simulink model "tip_assist_lib_support_pfw_latch_concepting"  (Simulink 9.0)
settings: Solver=VariableStepAuto  StartTime=0.0  StopTime=10.0  RelTol=1e-3
settings Model: Creator=CurriSD  LastModifiedBy=CurriSD
settings DataIOCC: SaveFormat=Dataset
settings OptimizationCC: LifeSpan=auto
settings DebuggingCC: UnderspecifiedInitializationDetection=Simplified  MergeDetectMultiDrivingBlocksExec=error  SFUnexpectedBacktrackingDiag=error  SFNoUnconditionalDefaultTransitionDiag=error  SFExecutionAtInitializationDiag=warning
settings HardwareCC: ProdBitPerPointer=64  ProdBitPerSizeT=64  ProdBitPerPtrDiffT=64  ProdLargestAtomicFloat=Float  ProdIntDivRoundTo=Zero  ProdEndianess=LittleEndian  ProdWordSize=64  ProdHWDeviceType=Intel->x86-64 (Windows64)
settings ModelReferenceCC: PropagateSignalLabelsOutOfModel=on
settings CodeAppCC: StateflowObjectComments=off
settings GRTTargetCC: TargetLangStandard=C99 (ISO)
settings ConfigComp: CovMetricSettings=dwe  CovHtmlReporting=off  CovSaveCumulativeToWorkspaceVar=off  CovSaveSingleToWorkspaceVar=off  CovExternalEMLEnable=on

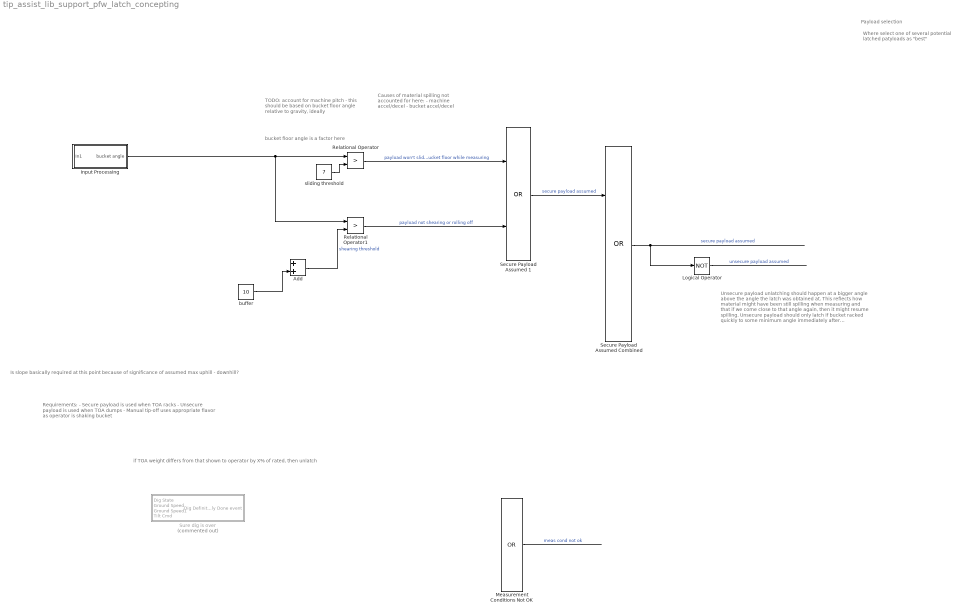
== system tip_assist_lib_support_pfw_latch_concepting ==
  note: if TOA weight differs from that shown to operator by X% of rated, then unlatch
  note: Is slope basically required at this point because of significance of assumed max uphill - downhill?
  note: Unsecure payload unlatching should happen at a bigger angle above the angle the latch was obtained at.  This reflects how material might have been still spilling when measuring and that if we come close to that angle again, then it might resume spilling.
      |
      | Unsecure payload should only latch if bucket racked quickly to some minimum angle immediately after measurement.  Otherwise, payload could still be falling out.
  note: Where select one of several potential latched patyloads as "best"
  note: Payload selection
  note: Requirements:
      | - Secure payload is used when TOA racks
      | - Unsecure payload is used when TOA dumps
      | - Manual tip-off uses appropriate flavor as operator is shaking bucket
  note: bucket floor angle is a factor here
  note: Causes of material spilling not accounted for here:
      | - machine accel/decel
      | - bucket accel/decel
  note: TODO: account for machine pitch - this should be based on bucket floor angle relative to gravity, ideally
  Add : Sum
  Input Processing : Subsystem
  Logical Operator : Logic  Operator=NOT  AllPortsSameDT=off  OutDataTypeStr=boolean
  Measurement Conditions Not OK : Logic  Operator=OR  Inputs=5  AllPortsSameDT=off  OutDataTypeStr=boolean
  Relational Operator : RelationalOperator  Operator=>  OutDataTypeStr=boolean  RndMeth=Simplest
  Relational Operator1 : RelationalOperator  Operator=>  OutDataTypeStr=boolean  RndMeth=Simplest
  Secure Payload Assumed 1 : Logic  Operator=OR  AllPortsSameDT=off  OutDataTypeStr=boolean
  Secure Payload Assumed Combined : Logic  Operator=OR  AllPortsSameDT=off  OutDataTypeStr=boolean
  Sure dig is over : Subsystem  Commented=on
  buffer : Constant  Value=10
  sliding threshold : Constant  Value=7
  wires:
  Measurement Conditions Not OK/1 -> ?  "meas cond not ok"
  Secure Payload Assumed Combined/1 -> Logical Operator/1  "secure payload assumed"
  Logical Operator/1 -> ?  "unsecure payload assumed"
  Relational Operator/1 -> Secure Payload Assumed 1/1  "payload won't slide out against bucket floor while measuring"
  Input Processing/1(bucket angle) -> Relational Operator1/1, Relational Operator/1
  sliding threshold/1 -> Relational Operator/2
  ? -> Measurement Conditions Not OK/1  "external force such as ground"
  ? -> Measurement Conditions Not OK/2  "digging"
  ? -> Measurement Conditions Not OK/3  "might be stalled"
  ? -> Add/1  "last angle of immediately prior dump cmd"
  Relational Operator1/1 -> Secure Payload Assumed 1/2  "payload not shearing or rolling off"
  buffer/1 -> Add/2
  Add/1 -> Relational Operator1/2  "shearing threshold"
  Secure Payload Assumed 1/1 -> Secure Payload Assumed Combined/1  "secure payload assumed"
  ? -> Secure Payload Assumed Combined/2  "bucket is racked"
  ? -> Measurement Conditions Not OK/4  "tilt or lift cmd"
  ? -> Measurement Conditions Not OK/5  "unlatch trigger set"

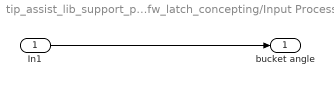
== system tip_assist_lib_support_pfw_latch_concepting/Input Processing ==
  In1 : Inport
  bucket angle : Outport
  wires:
  In1/1 -> bucket angle/1

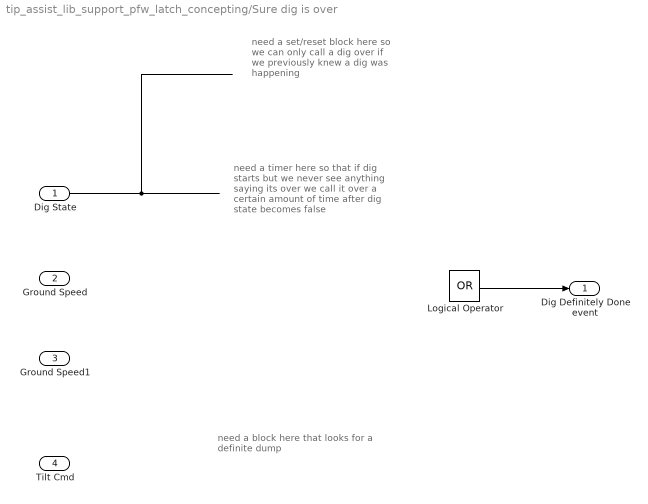
== system tip_assist_lib_support_pfw_latch_concepting/Sure dig is over ==
  note: need a set/reset block here so we can only call a dig over if we previously knew a dig was happening
  note: need a timer here so that if dig starts but we never see anything saying its over we call it over a certain amount of time after dig state becomes false
  note: need a block here that looks for a definite dump
  Dig State : Inport
  Ground Speed : Inport  Port=2
  Ground Speed1 : Inport  Port=3
  Tilt Cmd : Inport  Port=4
  Logical Operator : Logic  Operator=OR  AllPortsSameDT=off  OutDataTypeStr=boolean
  Dig Definitely Done event : Outport
  wires:
  Dig State/1 -> ?
  Logical Operator/1 -> Dig Definitely Done event/1
